simulink model "Homodyne_Tranceiver_v3"  (R2026b)
settings: Solver=VariableStepAuto  StopTime=0.001
undefined symbols (not defined in the file): S, sparameters
libraries: simrfV2elements x10, simrfV2util1 x4, fl_lib x3, nesl_utility x3, commutil2 x1, simrfV2_lib x1, slpidlib x1, simrfV2sources1 x1, ee_lib x1, simulink_extras x1
settings Model: Creator=dylan  LastModifiedBy=dylan
settings SimscapeCC: SimscapeLogType=all  SimscapeNominalValues="[{\"value\":\"1\",\"unit\":\"A\"},{\"value\":\"1\",\"unit\":\"bar\"},{\"value\":\"1\",\"unit\":\"cm^2\"},{\"value\":\"1\",\"unit\":\"cm^3/s\"},{\"value\":\"1\",\"unit\":\"kJ/kg\"},{\"value\":\"1\",\"unit\":\"kW\"},{\"value\":\"1\",\"unit\":\"l\"},{\"value\":\"1\",\"unit\":\"N\"},{\"value\":\"1\",\"unit\":\"N*m\"},{\"value\":\"1\",\"unit\":\"V\"},{\"value\":\"0.001\",\"unit\":\"Wb\"}]"  SimscapeUseEnergyAccounting=off

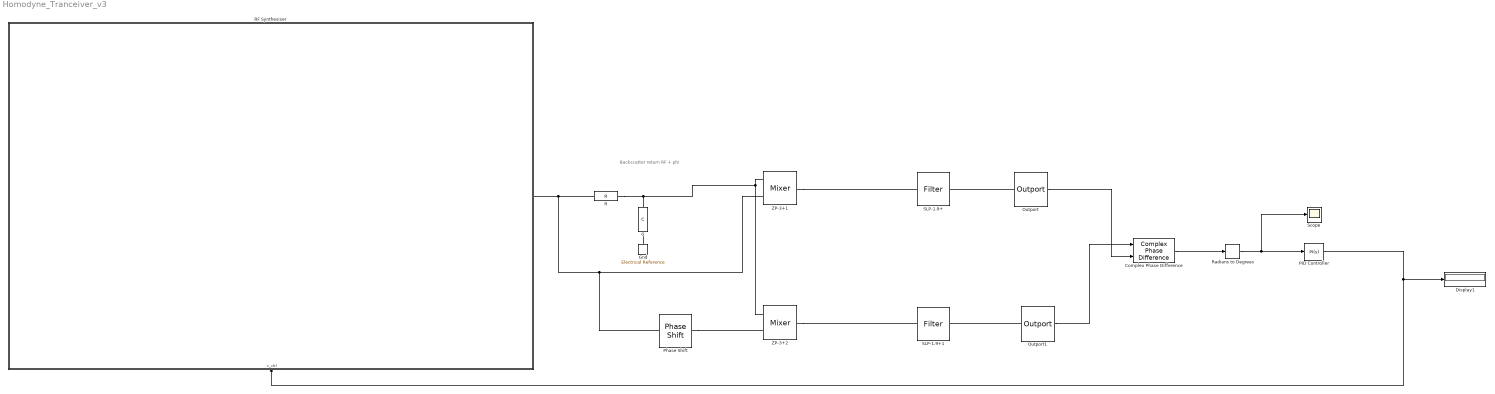
== system Homodyne_Tranceiver_v3 ==
  note: Backscatter return RF + phi
  C : simrfV2elements/C  classname=capacitor  Capacitance=139 pF
  Complex Phase Difference : commutil2/Complex Phase Difference
  Display1 : Display
  Gnd : simrfV2_lib/Elements/Electrical Reference
      settings: LibrarySourceBlock=simrfV2elements/Gnd
  Outport : simrfV2util1/Outport  SensorType=Ideal voltage  OutputFormat=Complex Baseband  CarrierFreq=0 MHz  ZL=Inf  AddNoise=off  InternalGrounding=on  StepSize=1e-09 s  AutoStep=on  HalfPolyphaseLength=12
  Outport1 : simrfV2util1/Outport  SensorType=Ideal voltage  OutputFormat=Complex Baseband  CarrierFreq=0 MHz  ZL=Inf  AddNoise=off  InternalGrounding=on  StepSize=1e-09 s  AutoStep=on  HalfPolyphaseLength=12
  PID Controller : slpidlib/PID Controller  Controller=PI  Form=Parallel  TimeDomain=Continuous-time  UseExternalTs=off  SampleTime=-1  IntegratorMethod=Forward Euler  FilterMethod=Forward Euler  ControllerParametersSource=internal  P=0.01  I=600  UseKiTs=off  D=0  UseExternalDerivativeSource=off  N=100  UseFilter=on  TunerSelectOption=Transfer Function Based (PID Tuner App)  InitialConditionSource=internal  InitialConditionForIntegrator=4  InitialConditionForFilter=0  DifferentiatorICPrevScaledInput=0  ExternalReset=none  TrackingMode=off  Kt=1  LimitOutput=on  SatLimitsSource=internal  UpperSaturationLimit=16  LowerSaturationLimit=1  LinearizeAsGain=on  AntiWindupMode=clamping  Kb=1  LimitIntegrator=off  UpperIntegratorSaturationLimit=inf  LowerIntegratorSaturationLimit=-inf  POutMin=[]  POutMax=[]  IOutMin=[]  IOutMax=[]  DOutMin=[]  DOutMax=[]  NOutMin=[]  NOutMax=[]  SumOutMin=[]  SumOutMax=[]  SaturationOutMin=[]  SaturationOutMax=[]  PParamMin=[]  PParamMax=[]  IParamMin=[]  IParamMax=[]  DParamMin=[]  DParamMax=[]  NParamMin=[]  NParamMax=[]  KbParamMin=[]  KbParamMax=[]  KtParamMin=[]  KtParamMax=[]  KbOutMin=[]  KbOutMax=[]  KtOutMin=[]  KtOutMax=[]  IntegratorOutMin=[]  IntegratorOutMax=[]  FilterOutMin=[]  FilterOutMax=[]  SumI1OutMin=[]  SumI1OutMax=[]  SumI2OutMin=[]  SumI2OutMax=[]  SumI3OutMin=[]  SumI3OutMax=[]  SumI4OutMin=[]  SumI4OutMax=[]  SumDOutMin=[]  SumDOutMax=[]  DifferentiatorOutMin=[]  DifferentiatorOutMax=[]  FilterDiffOutCoefMin=[]  FilterDiffOutCoefMax=[]  ReciprocalOutMin=[]  ReciprocalOutMax=[]  SumDenOutMin=[]  SumDenOutMax=[]  SumNumOutMin=[]  SumNumOutMax=[]  DivideOutMin=[]  DivideOutMax=[]  UdiffTsProdOutMin=[]  UdiffTsProdOutMax=[]  NTsProdOutMin=[]  NTsProdOutMax=[]  UintegralTsProdOutMin=[]  UintegralTsProdOutMax=[]  UngainTsProdOutMin=[]  UngainTsProdOutMax=[]  ClampingZeroOutDataTypeStr=Inherit: Inherit via back propagation  ClampingZeroOutMin=[]  ClampingZeroOutMax=[]  FilterDenConstantOutDataTypeStr=Inherit: Inherit via back propagation  FilterDenConstantOutMin=[]  FilterDenConstantOutMax=[]  PCopyOutDataTypeStr=Inherit: Inherit via back propagation  PCopyOutMin=[]  PCopyOutMax=[]  NCopyOutDataTypeStr=Inherit: Inherit via back propagation  NCopyOutMin=[]  NCopyOutMax=[]  IntegratorContinuousStateAttributes=''  IntegratorStateMustResolveToSignalObject=off  IntegratorRTWStateStorageClass=Auto  FilterContinuousStateAttributes=''  FilterStateMustResolveToSignalObject=off  FilterRTWStateStorageClass=Auto  ParallelPVariant=InternalParameters  IdealPVariant=Disabled  IVariant=InternalParameters  DVariant=Disabled  IntegratorVariant=Continuous  SatVariant=Enabled  AWVariant=ContClampingParallel  PCopyVariant=Disabled  TRVariant=Disabled  FdbkBlocksVariant=Forward  IdealPFdbkVariant=Disabled  SatFdbkVariant=Disabled  DerivativeFilterVariant=Disabled  NVariant=Disabled  NCopyVariant=Disabled_SignalSpec  FilterICVariant=Disabled  IntegratorICVariant=InternalICs  ExternalResetVariant=Disabled  TRSumVariant=Passthrough  SumFdbkVariant=Disabled  SumVariant=Sum_PI  TsampFilterVariant=InternalTs  TsampNgainVariant=Passthrough  TsampIntegralVariant=Disabled_SignalSpec  ExternalSaturationOutDataTypeStr=Inherit: Same as second input  DerivativeSourceVariant=Disabled  PreIntVariant=InternalPreInt
  Phase Shift : simrfV2elements/Phase Shift  PhaseShift=90 deg  InternalGrounding=on  PCBConvertable=on  PCBObjDesign={'design(phaseShifter,<DesignFreq>,''PhaseShift'',convert2Deg(<PhaseShift>,<PhaseShift_unit>))'}  PCBObjAllowed={{'phaseShifter'}}  PCBObjReroute={cell(1,0)}
  R : simrfV2elements/R  classname=resistor  Resistance=50 Ohm  AddNoise=on
  RF Synthesiser : Subsystem
      settings: PortSchema="{\"entries\":[{\"content\":{\"sides\":[{\"content\":{},\"type\":\"ConnectorPlacement.EquallySpacedRectSide\",\"uuid\":\"860778b0-137a-41ae-b7e0-f3ff562ae158\"},{\"content\":{\"connectorIds\":[\"RConn1\"],\"side\":\"RIGHT\"},\"type\":\"ConnectorPlacement.EquallySpacedRectSide\",\"uuid\":\"3be3f155-9c00-40bd-a560-b966d1cb54b3\"},{\"content\":{\"side\":\"TOP\"},\"type\":\"ConnectorPlacement.EquallySpacedRectSide\",\"uuid\":\"ab173a85-9f9a-436e-93c4-3cbd30c66835\"},{\"content\":{\"connectorIds\":[\"In1\"],\"side\":\"BOTTOM\"},\"type\":\"ConnectorPlacement.EquallySpacedRectSide\",\"uuid\":\"8e8f3058-61e1-4d47-8949-bf2a57e4e299\"}]},\"type\":\"ConnectorPlacement.EquallySpacedConnector\",\"uuid\":\"06351b81-de3c-49f3-a1c6-e9451bbace4c\"}],\"packageUris\":[\"http://schema.mathworks.com/mf0/Connector/R2020b\"],\"version\":\"1.0\"}"
  Radians to Degrees : simulink_extras/Transformations/Radians to Degrees
  SLP-1.9+ : simrfV2elements/Filter  classname=filter  DesignMethod=Butterworth  ResponseType=Lowpass  Implementation=LC Tee  ImplementationIdeal=Constant per carrier  ImplementationRational=Transfer function  UseFilterOrder=off  FilterOrder=3  PassFreq_lp=2.5 MHz  PassFreq_hp=2 GHz  PassFreq_bp=[2 3] GHz  PassFreq_bs=[1 4] GHz  PassAtten=10*log10(2)  StopFreq_lp=4.7 MHz  StopFreq_hp=1 GHz  StopFreq_bp=[1.5 3.5] GHz  StopFreq_bs=[2.1 2.9] GHz  StopAtten=40  Rsrc=50  Rload=50  AutoImpulseLength=on  ImpulseLength=1e-10 s  InternalGrounding=on  PlotFuncLeft=Voltage transfer  PlotLeftForm=Magnitude (dB)  PlotRightOnVT=None  PlotRightNoTD=None  PlotRightNoGD=None  PlotRightNoIR=None  PlotRightNoSR=None  PlotRightForm=Magnitude (dB)  FreqPoints=logspace(0,10,101)  Freq_unit=Hz  TimePoints=linspace(0,1,1e6+1)  Time_unit=s  XaxisScale=Linear  YaxisScale=Linear  needRedraw=0
  SLP-1.9+1 : simrfV2elements/Filter  classname=filter  DesignMethod=Butterworth  ResponseType=Lowpass  Implementation=LC Tee  ImplementationIdeal=Constant per carrier  ImplementationRational=Transfer function  UseFilterOrder=off  FilterOrder=3  PassFreq_lp=2.5 MHz  PassFreq_hp=2 GHz  PassFreq_bp=[2 3] GHz  PassFreq_bs=[1 4] GHz  PassAtten=10*log10(2)  StopFreq_lp=4.7 MHz  StopFreq_hp=1 GHz  StopFreq_bp=[1.5 3.5] GHz  StopFreq_bs=[2.1 2.9] GHz  StopAtten=40  Rsrc=50  Rload=50  AutoImpulseLength=on  ImpulseLength=1e-10 s  InternalGrounding=on  PlotFuncLeft=Voltage transfer  PlotLeftForm=Magnitude (dB)  PlotRightOnVT=None  PlotRightNoTD=None  PlotRightNoGD=None  PlotRightNoIR=None  PlotRightNoSR=None  PlotRightForm=Magnitude (dB)  FreqPoints=logspace(0,10,101)  Freq_unit=Hz  TimePoints=linspace(0,1,1e6+1)  Time_unit=s  XaxisScale=Linear  YaxisScale=Linear  needRedraw=0
  Scope : Scope
      settings: ActiveDisplayYMinimum=66.593123452666475  ActiveDisplayYMaximum=191.8815425426173
  ZP-3+1 : simrfV2elements/Mixer  classname=mixer  Source_linear_gain=Available power gain  linear_gain=-4.7 dB  Zin=50  Zout=50  ZLO=Inf  Poly_Coeffs=[0 1]  IPType=Input  IP2=Inf dBm  IP3=Inf dBm  P1dB=Inf dBm  Psat=Inf dBm  Gcomp=Inf dBm  NF=0  InternalGrounding=on
  ZP-3+2 : simrfV2elements/Mixer  classname=mixer  Source_linear_gain=Available power gain  linear_gain=-4.7 dB  Zin=50  Zout=50  ZLO=Inf  Poly_Coeffs=[0 1]  IPType=Input  IP2=Inf dBm  IP3=Inf dBm  P1dB=Inf dBm  Psat=Inf dBm  Gcomp=Inf dBm  NF=0  InternalGrounding=on
  wires:
  PID Controller/1 -> RF Synthesiser/1(v_ctrl), Display1/1
  Outport/1 -> Complex Phase Difference/2
  Outport1/1 -> Complex Phase Difference/1
  Complex Phase Difference/1 -> Radians to Degrees/1
  Radians to Degrees/1 -> Scope/1, PID Controller/1
  connections:
  ZP-3+1/RConn1 -- SLP-1.9+/LConn1
  Outport/LConn1 -- SLP-1.9+/RConn1
  RF Synthesiser/RConn1 -- R/LConn1 -- Phase Shift/LConn1 -- ZP-3+1/LConn2
  Phase Shift/RConn1 -- ZP-3+2/LConn2
  ZP-3+2/RConn1 -- SLP-1.9+1/LConn1
  Outport1/LConn1 -- SLP-1.9+1/RConn1
  ZP-3+1/LConn1 -- C/LConn1 -- R/RConn1 -- ZP-3+2/LConn1
  Gnd/LConn1 -- C/RConn1

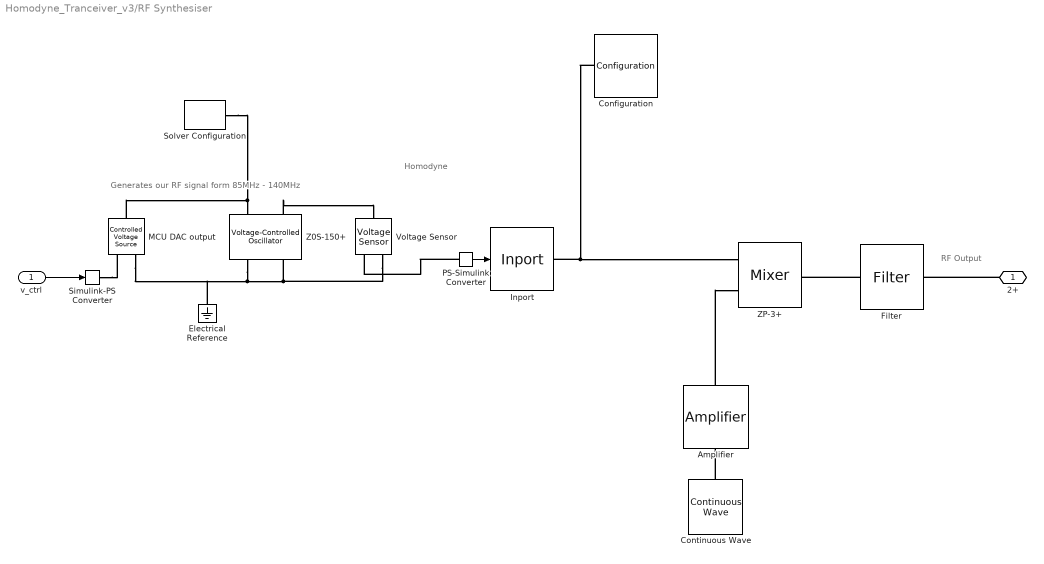
== system Homodyne_Tranceiver_v3/RF Synthesiser ==
  note: RF Output
  note: Homodyne
  note: Generates our RF signal form 85MHz - 140MHz
  v_ctrl : Inport
  Amplifier : simrfV2elements/Amplifier  classname=amplifier  DataSource=Data file  File=unitygain.s2p  isNetworkObj=off  NetworkObject=sparameters('default.s2p')  Paramtype=S-parameters  Sparam=[0 0;1 0]  SparamFreq=1e9 Hz  SparamZ0=50  isRationalObj=off  RationalObject=rational('unitygain.s2p', TendsToZero=false)  Residues=0  Poles=0  DF={0 0; 1 0}  Source_linear_gain=Available power gain  linear_gain=7 dB  AmAmAmPmTable=[-25,5,-1;-10,20,-2;0,27,5;5,28,12]  Zin=50  Zout=50  Poly_Coeffs=[0 1]  IPType=Output  IP2=inf dBm  IP3=inf dBm  P1dB=inf dBm  Psat=inf dBm  Gcomp=inf dBm  InternalGrounding=on  SourceFreq=Extracted from data source  PlotFreq=[1e9:1e6:3e9] Hz  PlotType=X-Y plane  YParam1=S(1,1)  YFormat1=Magnitude (dB)  YParam2=None  YFormat2=Magnitude (dB)  YOption=Linear  XOption=Linear  SparamRepresentation=Time domain  FitTol=-40  FitOpt=Fit individually  MaxPoles=48  AutoImpulseLength=on  ImpulseLength=1e-10 s  MagModeling=off  AddNoise=on  NoiseType=Noise figure  NoiseDist=White  NF=0  MinNF=0  Gopt=0  RN=0  CarrierFreq=0 Hz  NoiseAutoImpulseLength=on  NoiseImpulseLength=1e-10 s  ConstS21NL=off  OpFreq=1 GHz  SetOpFreqAsMaxS21=off
  Configuration : simrfV2util1/Configuration  AutoFreq=on  Tones=[0] Hz  Harmonics=[7]  NormalizeCarrierPower=on  SolverType=Auto  UseCCode=on  StepSize=1 ns  AddNoise=on  defaultRNG=on  Seed=0  Temperature=290.0 K  SolverDelFlag=0  AbsTol=1e-6  RelTol=1e-3  MaxIter=10  ErrorEstimationType=2-norm over all variables  EnableInterpFilter=on  HiddenFIRfilterControllerParam=on  SmallSignalApprox=off  AllSimFreqs=on  SimFreqs=[] Hz  SimFreqsInternal=[]  SamplesPerFrame=1
  Continuous Wave : simrfV2sources1/Continuous Wave  CWSourceType=Ideal voltage  Z0=0  IVoltage=1.782 V  ICurrent=0 A  MagPower=0 W  QVoltage=0 V  QCurrent=0 A  AnglePower=0  CarrierFreq=75 MHz  AddPhaseNoise=off  PhaseNoiseOffset=1  PhaseNoiseLevel=-Inf  AutoImpulseLength=on  ImpulseLength=1e-10 s  InternalGrounding=on
  Electrical Reference : fl_lib/Electrical/Electrical Elements/Electrical Reference
  Filter : simrfV2elements/Filter  classname=filter  DesignMethod=Butterworth  ResponseType=Lowpass  Implementation=LC Tee  ImplementationIdeal=Constant per carrier  ImplementationRational=Transfer function  UseFilterOrder=off  FilterOrder=3  PassFreq_lp=90 MHz  PassFreq_hp=2 GHz  PassFreq_bp=[2 3] GHz  PassFreq_bs=[1 4] GHz  PassAtten=10*log10(2)  StopFreq_lp=157 MHz  StopFreq_hp=1 GHz  StopFreq_bp=[1.5 3.5] GHz  StopFreq_bs=[2.1 2.9] GHz  StopAtten=40  Rsrc=50  Rload=50  AutoImpulseLength=on  ImpulseLength=1e-10 s  InternalGrounding=on  PlotFuncLeft=Voltage transfer  PlotLeftForm=Magnitude (dB)  PlotRightOnVT=None  PlotRightNoTD=None  PlotRightNoGD=None  PlotRightNoIR=None  PlotRightNoSR=None  PlotRightForm=Magnitude (dB)  FreqPoints=logspace(0,10,101)  Freq_unit=Hz  TimePoints=linspace(0,1,1e6+1)  Time_unit=s  XaxisScale=Linear  YaxisScale=Linear  needRedraw=0
  Inport : simrfV2util1/Inport  SimulinkInputSignalType=Ideal voltage  CarrierFreq=0 MHz  ZS=0  UseSqWave=off  NumCoeff=10  Bias=0  DutyCyc=50  AddNoise=off  InternalGrounding=on
  MCU DAC output : fl_lib/Electrical/Electrical Sources/Controlled Voltage Source
  PS-Simulink Converter : nesl_utility/PS-Simulink Converter  PhysicalDomain=network_engine_domain  SubClassName=ps_output  LeftPortType=input  RightPortType=output  PseudoPeriodic=off  Frequencies=[]  VectorFormat=inherit  Unit=inherit  AffineConversion=off
  Simulink-PS Converter : nesl_utility/Simulink-PS Converter  PhysicalDomain=network_engine_domain  SubClassName=ps_input  LeftPortType=input  RightPortType=output  PseudoPeriodic=off  Frequencies=[]  NoiseDistribution=none  NoiseParameters=[]  Unit=V  AffineConversion=off  FilteringAndDerivatives=filter  SimscapeFilterOrder=1  InputFilterTimeConstant=1e-7  UdotUserProvided=0
  Solver Configuration : nesl_utility/Solver Configuration  PhysicalDomain=network_engine_domain  SubClassName=solver  LeftPortType=input  RightPortType=generic  Tones=[]  Harmonics=[]  SimulateNoise=off  Profile=off  UseLocalSampling=off  EnableSwitchedLinearOptims=on  FrequencyDomain=off  UseCCode=off  RelTol=0.001  AbsTol=0.001  MinStep=1e-09  ToWorkspace=off  RevertToSquareIcSolve=off  NumHomotopyIterations=100  PhasorMode=off  PhasorModeNumHarmonics=1  ConsistencySolver=NEWTON_XTOL_AFTER_FTOL  CanonicalOrdering=CANONICAL  OptimizeIntermediates=OPTIMIZED  MulticoreSolverChoice=BACKWARD_EULER  IndexReductionMethod=DerivativeReplacement  DoDC=off  ResidualTolerance=1e-09  ConsistencyTolSource=GLOBAL  ConsistencyAbsTol=0.001  ConsistencyRelTol=0.001  ConsistencyTolFactor=0.001  UseLocalSolver=off  LocalSolverChoice=NE_BACKWARD_EULER_ADVANCER  ResolveIndetEquations=on  FunctionEvalNumThread=1  LocalSolverSampleTime=0.001  DoFixedCost=off  MaxNonlinIter=3  MaxModeIter=2  ComputeImpulses=off  ImpulseIterations=2  LinearAlgebra=auto  LinearAlgebraNumThread=0  EquationFormulation=NE_TIME_EF  DelaysMemoryBudget=1024  AutomaticFiltering=on  FilteringTimeConstant=0.001  PartitionStorageMethod=AS_NEEDED  PartitionMemoryBudget=1024  PartitionMethod=BALANCED  MultibodyUseLocalSolver=off  MultibodyLocalSolverChoice=ODE1  MultibodyLocalSolverSampleTime=0.001
  Voltage Sensor : fl_lib/Electrical/Electrical Sensors/Voltage Sensor
  Z0S-150+ : ee_lib/Integrated Circuits/Voltage-Controlled Oscillator  tabulated=ee.enum.ic.vcoFrequencyDependence.linear  f_nom=75 MHz  v_nom=1 V  df_dv=5800000 Hz/V  v_min=1 V  v_max=16 V  v_vec=[0, .2, .4, .6, .8, 1] V  f_vec=[-1000, -329, -51, 162, 342, 500] Hz  v_out=1.782 V  r_in=inf Ohm  r_out=50 Ohm  model_dynamics=ee.enum.ic.vcoDynamics.no  time_constant=1.59e-6 s  f_ini=75 MHz
  ZP-3+ : simrfV2elements/Mixer  classname=mixer  Source_linear_gain=Available power gain  linear_gain=-4.7 dB  Zin=50  Zout=50  ZLO=Inf  Poly_Coeffs=[0 1]  IPType=Input  IP2=Inf dBm  IP3=Inf dBm  P1dB=Inf dBm  Psat=Inf dBm  Gcomp=Inf dBm  NF=4.7  InternalGrounding=on
  2+ : PMIOPort  Side=Right
  wires:
  PS-Simulink Converter/1 -> Inport/1
  v_ctrl/1 -> Simulink-PS Converter/1
  connections:
  Z0S-150+/LConn2 -- Voltage Sensor/LConn1
  MCU DAC output/LConn1 -- Solver Configuration/RConn1 -- Z0S-150+/LConn1
  Configuration/LConn1 -- ZP-3+/LConn1 -- Inport/RConn1
  Simulink-PS Converter/RConn1 -- MCU DAC output/RConn1
  Z0S-150+/RConn1 -- Electrical Reference/LConn1 -- MCU DAC output/RConn2 -- Voltage Sensor/RConn2 -- Z0S-150+/RConn2
  PS-Simulink Converter/LConn1 -- Voltage Sensor/RConn1
  Filter/LConn1 -- ZP-3+/RConn1
  Amplifier/RConn1 -- ZP-3+/LConn2
  2+/RConn1 -- Filter/RConn1
  Continuous Wave/LConn1 -- Amplifier/LConn1
